simulink model "MRAC_PID_unblance_noposition"  (R2024a)
settings: Solver=FixedStepAuto  StartTime=0.0  StopTime=30  FixedStep=0.001  RelTol=1e-3
values from neighbouring files (symbols this model uses):
  B = [ ... (first row only)    [untitled1.m]
  cM = 2.925e-9    (= 2.925e-09)    [untitled1.m]
  CR = 80.584    [untitled1.m]
  cT = 1.4865e-7    (= 1.4865e-07)    [untitled1.m]
  d_x = 0.08257    [untitled1.m]
  d_y = 0.13505    [untitled1.m]
  g = 9.81    [untitled1.m]
  Ix = 0.0095    [untitled1.m]
  Iy = 0.0095    [untitled1.m]
  Iz = 0.019    [untitled1.m]
  K = cM/cT    (= 0.0196770938446)    [untitled1.m]
  Kposi = 0.1    [untitled1.m]
  Kposp = 1.5    [untitled1.m]
  Kvd = 0    [untitled1.m]
  Kvi = 0    [untitled1.m]
  Kvp = 1    [untitled1.m]
  Kvxd = 10    [untitled1.m]
  Kvxi = 0.001    [untitled1.m]
  Kvxp = 5    [untitled1.m]
  Kvyd = 10    [untitled1.m]
  Kvyi = 0.001    [untitled1.m]
  Kvyp = 5    [untitled1.m]
  Kvzd = 0.1    [untitled1.m]
  Kvzi = 0.01    [untitled1.m]
  Kvzp = 10    [untitled1.m]
  M = inv(B)    [untitled1.m]
  m = 2    [untitled1.m]
  Tm = 0.03    [untitled1.m]
  wb = 976.2    [untitled1.m]
  x1 = d_x    (= 0.08257)    [untitled1.m]
  x2 = d_x    (= 0.08257)    [untitled1.m]
  x3 = -d_x    (= -0.08257)    [untitled1.m]
  x4 = -d_x    (= -0.08257)    [untitled1.m]
  y1 = d_y    (= 0.13505)    [untitled1.m]
  y2 = -d_y    (= -0.13505)    [untitled1.m]
  y3 = -d_y    (= -0.13505)    [untitled1.m]
  y4 = d_y    (= 0.13505)    [untitled1.m]
undefined symbols (not defined in the file or in its folder): magnitude
libraries: slpidlib x5
settings Model: Creator=user  LastModifiedBy=User
settings DataIOCC: ReturnWorkspaceOutputs=off

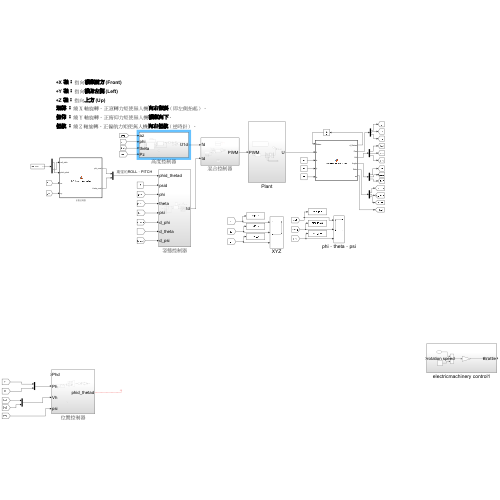
[thumbnail: Simulink's stored preview of the top-level diagram]
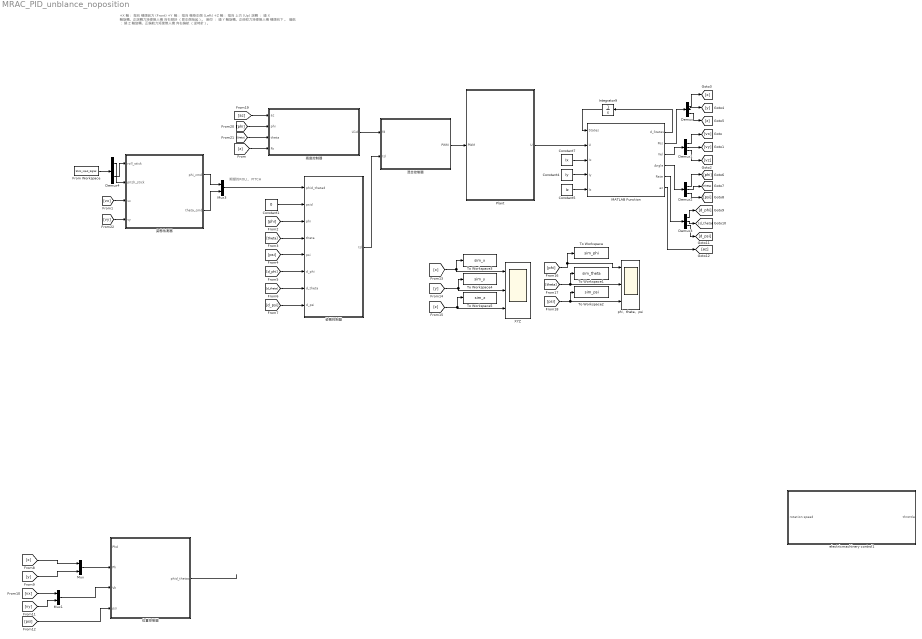
== system MRAC_PID_unblance_noposition ==
  note: +X 軸： 指向 機頭前方 (Front)
      | +Y 軸： 指向 機身左側 (Left)
      | +Z 軸： 指向 上方 (Up)
      | 滾轉 ： 繞 X 軸旋轉。正滾轉力矩使無人機 向右傾斜 （即左側抬起）。
      | 俯仰 ： 繞 Y 軸旋轉。正俯仰力矩使無人機 機頭向下 。
      | 偏航 ： 繞 Z 軸旋轉。正偏航力矩使無人機 向右偏航 （逆時針）。
  note: 期望的ROLL、PITCH
  Constant1 : Constant  Value=0
  Constant4 : Constant  Value=Iy
  Constant5 : Constant  Value=Iz
  Constant7 : Constant  Value=Ix
  Demux{,1..3} (4 alike) : Demux  Outputs=3
  Demux4 : Demux  Outputs=2
  From Workspace : FromWorkspace  VariableName=Stick_Input_Signal
  Integrator9 : Integrator  InitialCondition=zeros(12,1)
  MATLAB Function : MATLAB Function  TreatAsAtomicUnit=on
  Mux : Mux  Inputs=2
  Mux1 : Mux  Inputs=2
  Mux3 : Mux  Inputs=2
  Plant : Subsystem
  To Workspace : ToWorkspace  VariableName=sim_phi  SampleTime=-1
  To Workspace1 : ToWorkspace  VariableName=sim_theta  SampleTime=-1
  To Workspace2 : ToWorkspace  VariableName=sim_psi  SampleTime=-1
  To Workspace3 : ToWorkspace  VariableName=sim_x  SampleTime=-1
  To Workspace4 : ToWorkspace  VariableName=sim_y  SampleTime=-1
  To Workspace5 : ToWorkspace  VariableName=sim_z  SampleTime=-1
  XYZ : Scope  NumInputPorts=3
  electricmachinery control1 : Subsystem
  phi、theta、psi : Scope  NumInputPorts=3
  位置控制器 : Subsystem
  姿態估測器 : MATLAB Function  TreatAsAtomicUnit=on
  姿態控制器 : Subsystem
  混合控制器 : Subsystem
  高度控制器 : Subsystem
  wires:
  高度控制器/1(U1d) -> 混合控制器/1(fd)
  [z] -> 高度控制器/4(Pz)
  位置控制器/1(phid_thetad) -> ?
  Constant1/1 -> 姿態控制器/2(psid)
  [phi] -> 姿態控制器/3(phi)
  [theta] -> 姿態控制器/4(theta)
  [d_psi] -> 姿態控制器/8(d_psi)
  [psi] -> 姿態控制器/5(psi)
  [d_phi] -> 姿態控制器/6(d_phi)
  [d_theta] -> 姿態控制器/7(d_theta)
  姿態控制器/1(td) -> 混合控制器/2(td)
  Mux/1 -> 位置控制器/2(Ph)
  [x] -> Mux/1
  [y] -> Mux/2
  [vx] -> Mux1/1
  [vy] -> Mux1/2
  Mux1/1 -> 位置控制器/3(Vh)
  [psi] -> 位置控制器/4(psi)
  [y] -> To Workspace4/1, XYZ/2
  [x] -> To Workspace3/1, XYZ/1
  [z] -> To Workspace5/1, XYZ/3
  [phi] -> To Workspace/1, phi、theta、psi/1
  [theta] -> To Workspace1/1, phi、theta、psi/2
  [psi] -> To Workspace2/1, phi、theta、psi/3
  混合控制器/1(PWM) -> Plant/1(PWM)
  Constant5/1 -> MATLAB Function/5(Iz)
  Constant7/1 -> MATLAB Function/3(Ix)
  Constant4/1 -> MATLAB Function/4(Iy)
  MATLAB Function/1(d_States) -> Integrator9/1
  Integrator9/1 -> MATLAB Function/1(States)
  MATLAB Function/2(Pos) -> Demux/1
  Demux/1 -> [x]
  Demux/2 -> [y]
  Demux/3 -> [z]
  Demux1/2 -> [vy]
  MATLAB Function/3(Vel) -> Demux1/1
  Demux1/1 -> [vx]
  Demux1/3 -> [vz]
  MATLAB Function/4(Angle) -> Demux2/1
  Demux2/1 -> [phi]
  Demux2/2 -> [theta]
  Demux2/3 -> [psi]
  Demux3/1 -> [d_phi]
  Demux3/2 -> [d_theta]
  Demux3/3 -> [d_psi]
  MATLAB Function/5(Rate) -> Demux3/1
  Plant/1(U) -> MATLAB Function/2(U)
  姿態估測器/1(phi_cmd) -> Mux3/1
  Mux3/1 -> 姿態控制器/1(phid_thetad)
  MATLAB Function/6(az) -> [az]
  [az] -> 高度控制器/1(az)
  [phi] -> 高度控制器/2(phi)
  [theta] -> 高度控制器/3(theta)
  From Workspace/1 -> Demux4/1
  Demux4/1 -> 姿態估測器/2(pitch_stick)
  Demux4/2 -> 姿態估測器/1(roll_stick)
  [vx] -> 姿態估測器/3(vx)
  [vy] -> 姿態估測器/4(vy)
  姿態估測器/2(theta_cmd) -> Mux3/2

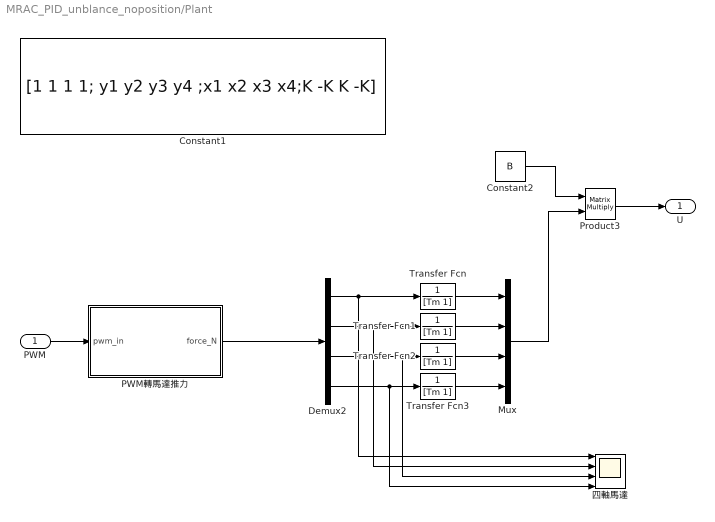
== system MRAC_PID_unblance_noposition/Plant ==
  PWM : Inport
  Constant1 : Constant  Value=[1 1 1 1; y1 y2 y3 y4 ;x1 x2 x3 x4;K -K K -K]
  Constant2 : Constant  Value=B
  Demux2 : Demux
  Mux : Mux
  PWM轉馬達推力 : MATLAB Function  TreatAsAtomicUnit=on
  Product3 : Product  Multiplication=Matrix(*)
  Transfer Fcn{,1..3} (4 alike) : TransferFcn  Denominator=[Tm 1]
  四軸馬達 : Scope  NumInputPorts=4
  U : Outport
  wires:
  Product3/1 -> U/1
  PWM/1 -> PWM轉馬達推力/1(pwm_in)
  Demux2/2 -> Transfer Fcn1/1, 四軸馬達/2
  Demux2/3 -> Transfer Fcn2/1, 四軸馬達/3
  PWM轉馬達推力/1(force_N) -> Demux2/1
  Demux2/4 -> 四軸馬達/4, Transfer Fcn3/1
  Demux2/1 -> Transfer Fcn/1, 四軸馬達/1
  Transfer Fcn1/1 -> Mux/2
  Transfer Fcn/1 -> Mux/1
  Transfer Fcn2/1 -> Mux/3
  Transfer Fcn3/1 -> Mux/4
  Mux/1 -> Product3/2
  Constant2/1 -> Product3/1

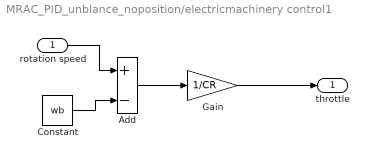
== system MRAC_PID_unblance_noposition/electricmachinery control1 ==
  rotation speed : Inport
  Add : Sum  Inputs=+-
  Constant : Constant  Value=wb
  Gain : Gain  Gain=1/CR
  throttle : Outport
  wires:
  Add/1 -> Gain/1
  rotation speed/1 -> Add/1
  Constant/1 -> Add/2
  Gain/1 -> throttle/1

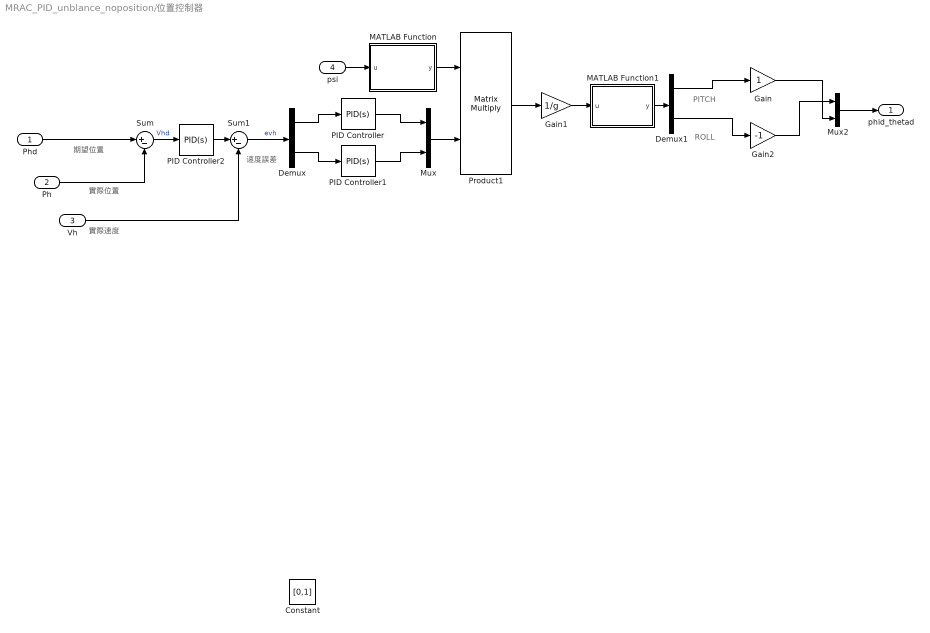
== system MRAC_PID_unblance_noposition/位置控制器 ==
  note: ROLL
  note: 期望位置
  note: 實際位置
  note: 實際速度
  note: 速度誤差
  note: PITCH
  Phd : Inport
  Ph : Inport  Port=2
  Vh : Inport  Port=3
  psi : Inport  Port=4
  Constant : Constant  Value=[0,1]
  Demux : Demux  Outputs=2
  Demux1 : Demux  Outputs=2
  Gain : Gain
  Gain1 : Gain  Gain=1/g
  Gain2 : Gain  Gain=-1
  MATLAB Function : MATLAB Function  TreatAsAtomicUnit=on
  MATLAB Function1 : MATLAB Function  TreatAsAtomicUnit=on
  Mux : Mux  Inputs=2
  Mux2 : Mux  Inputs=2
  PID Controller : slpidlib/PID Controller  Controller=PID  Form=Parallel  TimeDomain=Continuous-time  UseExternalTs=off  SampleTime=-1  IntegratorMethod=Forward Euler  FilterMethod=Forward Euler  ControllerParametersSource=internal  P=Kvxp  I=Kvxi  UseKiTs=off  D=Kvxd  UseExternalDerivativeSource=off  N=100  UseFilter=on  TunerSelectOption=Transfer Function Based (PID Tuner App)  InitialConditionSource=internal  InitialConditionForIntegrator=0  InitialConditionForFilter=0  DifferentiatorICPrevScaledInput=0  ExternalReset=none  TrackingMode=off  Kt=1  LimitOutput=off  SatLimitsSource=internal  UpperSaturationLimit=inf  LowerSaturationLimit=-inf  LinearizeAsGain=on  AntiWindupMode=none  Kb=1  LimitIntegrator=off  UpperIntegratorSaturationLimit=inf  LowerIntegratorSaturationLimit=-inf  POutMin=[]  POutMax=[]  IOutMin=[]  IOutMax=[]  DOutMin=[]  DOutMax=[]  NOutMin=[]  NOutMax=[]  SumOutMin=[]  SumOutMax=[]  SaturationOutMin=[]  SaturationOutMax=[]  PParamMin=[]  PParamMax=[]  IParamMin=[]  IParamMax=[]  DParamMin=[]  DParamMax=[]  NParamMin=[]  NParamMax=[]  KbParamMin=[]  KbParamMax=[]  KtParamMin=[]  KtParamMax=[]  KbOutMin=[]  KbOutMax=[]  KtOutMin=[]  KtOutMax=[]  IntegratorOutMin=[]  IntegratorOutMax=[]  FilterOutMin=[]  FilterOutMax=[]  SumI1OutMin=[]  SumI1OutMax=[]  SumI2OutMin=[]  SumI2OutMax=[]  SumI3OutMin=[]  SumI3OutMax=[]  SumI4OutMin=[]  SumI4OutMax=[]  SumDOutMin=[]  SumDOutMax=[]  DifferentiatorOutMin=[]  DifferentiatorOutMax=[]  FilterDiffOutCoefMin=[]  FilterDiffOutCoefMax=[]  ReciprocalOutMin=[]  ReciprocalOutMax=[]  SumDenOutMin=[]  SumDenOutMax=[]  SumNumOutMin=[]  SumNumOutMax=[]  DivideOutMin=[]  DivideOutMax=[]  UdiffTsProdOutMin=[]  UdiffTsProdOutMax=[]  NTsProdOutMin=[]  NTsProdOutMax=[]  UintegralTsProdOutMin=[]  UintegralTsProdOutMax=[]  UngainTsProdOutMin=[]  UngainTsProdOutMax=[]  ClampingZeroOutDataTypeStr=Inherit: Inherit via back propagation  ClampingZeroOutMin=[]  ClampingZeroOutMax=[]  FilterDenConstantOutDataTypeStr=Inherit: Inherit via back propagation  FilterDenConstantOutMin=[]  FilterDenConstantOutMax=[]  PCopyOutDataTypeStr=Inherit: Inherit via back propagation  PCopyOutMin=[]  PCopyOutMax=[]  NCopyOutDataTypeStr=Inherit: Inherit via back propagation  NCopyOutMin=[]  NCopyOutMax=[]  IntegratorContinuousStateAttributes=''  IntegratorStateMustResolveToSignalObject=off  IntegratorRTWStateStorageClass=Auto  FilterContinuousStateAttributes=''  FilterStateMustResolveToSignalObject=off  FilterRTWStateStorageClass=Auto  ParallelPVariant=InternalParameters  IdealPVariant=Disabled  IVariant=InternalParameters  DVariant=InternalParameters  IntegratorVariant=Continuous  SatVariant=Disabled  AWVariant=Passthrough  PCopyVariant=Disabled  TRVariant=Disabled  FdbkBlocksVariant=Forward  IdealPFdbkVariant=Disabled  SatFdbkVariant=Disabled  DerivativeFilterVariant=ContFilter  NVariant=InternalParameters  NCopyVariant=Disabled  FilterICVariant=InternalICsFilter  IntegratorICVariant=InternalICs  ExternalResetVariant=Disabled  TRSumVariant=Passthrough  SumFdbkVariant=Disabled  SumVariant=Sum_PID  TsampFilterVariant=InternalTs  TsampNgainVariant=Passthrough  TsampIntegralVariant=Disabled_SignalSpec  ExternalSaturationOutDataTypeStr=Inherit: Same as second input  DerivativeSourceVariant=ErrorSignal
  PID Controller1 : slpidlib/PID Controller  Controller=PID  Form=Parallel  TimeDomain=Continuous-time  UseExternalTs=off  SampleTime=-1  IntegratorMethod=Forward Euler  FilterMethod=Forward Euler  ControllerParametersSource=internal  P=Kvyp  I=Kvyi  UseKiTs=off  D=Kvyd  UseExternalDerivativeSource=off  N=100  UseFilter=on  TunerSelectOption=Transfer Function Based (PID Tuner App)  InitialConditionSource=internal  InitialConditionForIntegrator=0  InitialConditionForFilter=0  DifferentiatorICPrevScaledInput=0  ExternalReset=none  TrackingMode=off  Kt=1  LimitOutput=off  SatLimitsSource=internal  UpperSaturationLimit=inf  LowerSaturationLimit=-inf  LinearizeAsGain=on  AntiWindupMode=none  Kb=1  LimitIntegrator=off  UpperIntegratorSaturationLimit=inf  LowerIntegratorSaturationLimit=-inf  POutMin=[]  POutMax=[]  IOutMin=[]  IOutMax=[]  DOutMin=[]  DOutMax=[]  NOutMin=[]  NOutMax=[]  SumOutMin=[]  SumOutMax=[]  SaturationOutMin=[]  SaturationOutMax=[]  PParamMin=[]  PParamMax=[]  IParamMin=[]  IParamMax=[]  DParamMin=[]  DParamMax=[]  NParamMin=[]  NParamMax=[]  KbParamMin=[]  KbParamMax=[]  KtParamMin=[]  KtParamMax=[]  KbOutMin=[]  KbOutMax=[]  KtOutMin=[]  KtOutMax=[]  IntegratorOutMin=[]  IntegratorOutMax=[]  FilterOutMin=[]  FilterOutMax=[]  SumI1OutMin=[]  SumI1OutMax=[]  SumI2OutMin=[]  SumI2OutMax=[]  SumI3OutMin=[]  SumI3OutMax=[]  SumI4OutMin=[]  SumI4OutMax=[]  SumDOutMin=[]  SumDOutMax=[]  DifferentiatorOutMin=[]  DifferentiatorOutMax=[]  FilterDiffOutCoefMin=[]  FilterDiffOutCoefMax=[]  ReciprocalOutMin=[]  ReciprocalOutMax=[]  SumDenOutMin=[]  SumDenOutMax=[]  SumNumOutMin=[]  SumNumOutMax=[]  DivideOutMin=[]  DivideOutMax=[]  UdiffTsProdOutMin=[]  UdiffTsProdOutMax=[]  NTsProdOutMin=[]  NTsProdOutMax=[]  UintegralTsProdOutMin=[]  UintegralTsProdOutMax=[]  UngainTsProdOutMin=[]  UngainTsProdOutMax=[]  ClampingZeroOutDataTypeStr=Inherit: Inherit via back propagation  ClampingZeroOutMin=[]  ClampingZeroOutMax=[]  FilterDenConstantOutDataTypeStr=Inherit: Inherit via back propagation  FilterDenConstantOutMin=[]  FilterDenConstantOutMax=[]  PCopyOutDataTypeStr=Inherit: Inherit via back propagation  PCopyOutMin=[]  PCopyOutMax=[]  NCopyOutDataTypeStr=Inherit: Inherit via back propagation  NCopyOutMin=[]  NCopyOutMax=[]  IntegratorContinuousStateAttributes=''  IntegratorStateMustResolveToSignalObject=off  IntegratorRTWStateStorageClass=Auto  FilterContinuousStateAttributes=''  FilterStateMustResolveToSignalObject=off  FilterRTWStateStorageClass=Auto  ParallelPVariant=InternalParameters  IdealPVariant=Disabled  IVariant=InternalParameters  DVariant=InternalParameters  IntegratorVariant=Continuous  SatVariant=Disabled  AWVariant=Passthrough  PCopyVariant=Disabled  TRVariant=Disabled  FdbkBlocksVariant=Forward  IdealPFdbkVariant=Disabled  SatFdbkVariant=Disabled  DerivativeFilterVariant=ContFilter  NVariant=InternalParameters  NCopyVariant=Disabled  FilterICVariant=InternalICsFilter  IntegratorICVariant=InternalICs  ExternalResetVariant=Disabled  TRSumVariant=Passthrough  SumFdbkVariant=Disabled  SumVariant=Sum_PID  TsampFilterVariant=InternalTs  TsampNgainVariant=Passthrough  TsampIntegralVariant=Disabled_SignalSpec  ExternalSaturationOutDataTypeStr=Inherit: Same as second input  DerivativeSourceVariant=ErrorSignal
  PID Controller2 : slpidlib/PID Controller  Controller=PID  Form=Parallel  TimeDomain=Continuous-time  UseExternalTs=off  SampleTime=-1  IntegratorMethod=Forward Euler  FilterMethod=Forward Euler  ControllerParametersSource=internal  P=Kposp  I=Kposi  UseKiTs=off  D=0  UseExternalDerivativeSource=off  N=100  UseFilter=on  TunerSelectOption=Transfer Function Based (PID Tuner App)  InitialConditionSource=internal  InitialConditionForIntegrator=0  InitialConditionForFilter=0  DifferentiatorICPrevScaledInput=0  ExternalReset=none  TrackingMode=off  Kt=1  LimitOutput=off  SatLimitsSource=internal  UpperSaturationLimit=inf  LowerSaturationLimit=-inf  LinearizeAsGain=on  AntiWindupMode=none  Kb=1  LimitIntegrator=off  UpperIntegratorSaturationLimit=inf  LowerIntegratorSaturationLimit=-inf  POutMin=[]  POutMax=[]  IOutMin=[]  IOutMax=[]  DOutMin=[]  DOutMax=[]  NOutMin=[]  NOutMax=[]  SumOutMin=[]  SumOutMax=[]  SaturationOutMin=[]  SaturationOutMax=[]  PParamMin=[]  PParamMax=[]  IParamMin=[]  IParamMax=[]  DParamMin=[]  DParamMax=[]  NParamMin=[]  NParamMax=[]  KbParamMin=[]  KbParamMax=[]  KtParamMin=[]  KtParamMax=[]  KbOutMin=[]  KbOutMax=[]  KtOutMin=[]  KtOutMax=[]  IntegratorOutMin=[]  IntegratorOutMax=[]  FilterOutMin=[]  FilterOutMax=[]  SumI1OutMin=[]  SumI1OutMax=[]  SumI2OutMin=[]  SumI2OutMax=[]  SumI3OutMin=[]  SumI3OutMax=[]  SumI4OutMin=[]  SumI4OutMax=[]  SumDOutMin=[]  SumDOutMax=[]  DifferentiatorOutMin=[]  DifferentiatorOutMax=[]  FilterDiffOutCoefMin=[]  FilterDiffOutCoefMax=[]  ReciprocalOutMin=[]  ReciprocalOutMax=[]  SumDenOutMin=[]  SumDenOutMax=[]  SumNumOutMin=[]  SumNumOutMax=[]  DivideOutMin=[]  DivideOutMax=[]  UdiffTsProdOutMin=[]  UdiffTsProdOutMax=[]  NTsProdOutMin=[]  NTsProdOutMax=[]  UintegralTsProdOutMin=[]  UintegralTsProdOutMax=[]  UngainTsProdOutMin=[]  UngainTsProdOutMax=[]  ClampingZeroOutDataTypeStr=Inherit: Inherit via back propagation  ClampingZeroOutMin=[]  ClampingZeroOutMax=[]  FilterDenConstantOutDataTypeStr=Inherit: Inherit via back propagation  FilterDenConstantOutMin=[]  FilterDenConstantOutMax=[]  PCopyOutDataTypeStr=Inherit: Inherit via back propagation  PCopyOutMin=[]  PCopyOutMax=[]  NCopyOutDataTypeStr=Inherit: Inherit via back propagation  NCopyOutMin=[]  NCopyOutMax=[]  IntegratorContinuousStateAttributes=''  IntegratorStateMustResolveToSignalObject=off  IntegratorRTWStateStorageClass=Auto  FilterContinuousStateAttributes=''  FilterStateMustResolveToSignalObject=off  FilterRTWStateStorageClass=Auto  ParallelPVariant=InternalParameters  IdealPVariant=Disabled  IVariant=InternalParameters  DVariant=InternalParameters  IntegratorVariant=Continuous  SatVariant=Disabled  AWVariant=Passthrough  PCopyVariant=Disabled  TRVariant=Disabled  FdbkBlocksVariant=Forward  IdealPFdbkVariant=Disabled  SatFdbkVariant=Disabled  DerivativeFilterVariant=ContFilter  NVariant=InternalParameters  NCopyVariant=Disabled  FilterICVariant=InternalICsFilter  IntegratorICVariant=InternalICs  ExternalResetVariant=Disabled  TRSumVariant=Passthrough  SumFdbkVariant=Disabled  SumVariant=Sum_PID  TsampFilterVariant=InternalTs  TsampNgainVariant=Passthrough  TsampIntegralVariant=Disabled_SignalSpec  ExternalSaturationOutDataTypeStr=Inherit: Same as second input  DerivativeSourceVariant=ErrorSignal
  Product1 : Product  Multiplication=Matrix(*)
  Sum : Sum  Inputs=|+-
  Sum1 : Sum  Inputs=|+-
  phid_thetad : Outport
  wires:
  Gain1/1 -> MATLAB Function1/1(u)
  Demux/1 -> PID Controller/1
  Product1/1 -> Gain1/1
  PID Controller/1 -> Mux/1
  Demux/2 -> PID Controller1/1
  Sum1/1 -> Demux/1  "evh"
  Mux/1 -> Product1/2
  Sum/1 -> PID Controller2/1  "Vhd"
  MATLAB Function1/1(y) -> Demux1/1
  MATLAB Function/1(y) -> Product1/1
  PID Controller1/1 -> Mux/2
  Demux1/1 -> Gain/1
  Gain/1 -> Mux2/2
  Mux2/1 -> phid_thetad/1
  Ph/1 -> Sum/2
  Phd/1 -> Sum/1
  PID Controller2/1 -> Sum1/1
  Vh/1 -> Sum1/2
  Demux1/2 -> Gain2/1
  psi/1 -> MATLAB Function/1(u)
  Gain2/1 -> Mux2/1

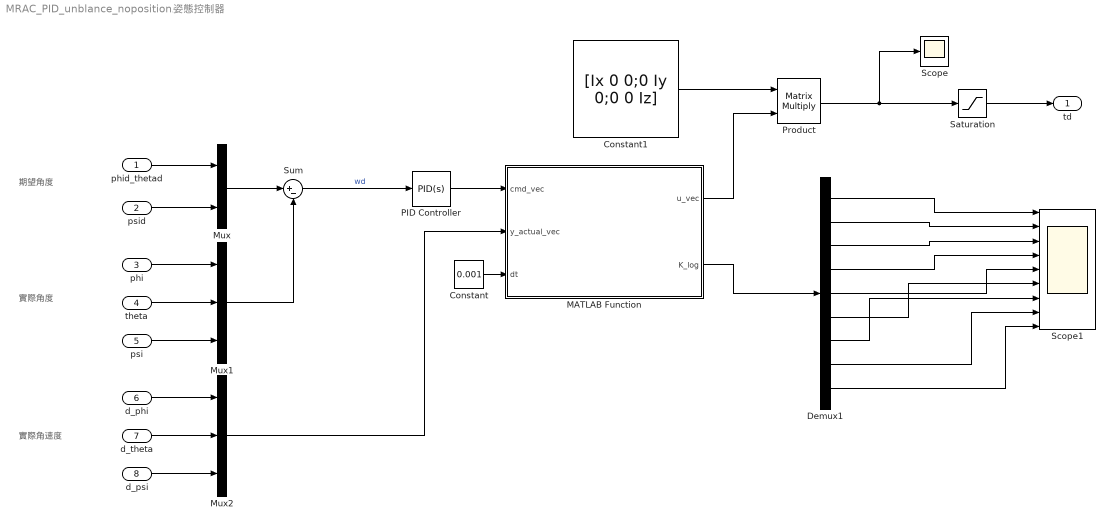
== system MRAC_PID_unblance_noposition/姿態控制器 ==
  note: 實際角速度
  note: 實際角度
  note: 期望角度
  phid_thetad : Inport
  psid : Inport  Port=2
  phi : Inport  Port=3
  theta : Inport  Port=4
  psi : Inport  Port=5
  d_phi : Inport  Port=6
  d_theta : Inport  Port=7
  d_psi : Inport  Port=8
  Constant : Constant  Value=0.001
  Constant1 : Constant  Value=[Ix 0 0;0 Iy 0;0 0 Iz]
  Demux1 : Demux  Outputs=9
  MATLAB Function : MATLAB Function  TreatAsAtomicUnit=on
  Mux : Mux  Inputs=2
  Mux1 : Mux  Inputs=3
  Mux2 : Mux  Inputs=3
  PID Controller : slpidlib/PID Controller  Controller=PID  Form=Parallel  TimeDomain=Continuous-time  UseExternalTs=off  SampleTime=-1  IntegratorMethod=Forward Euler  FilterMethod=Forward Euler  ControllerParametersSource=internal  P=Kvp  I=Kvi  UseKiTs=off  D=Kvd  UseExternalDerivativeSource=off  N=100  UseFilter=on  TunerSelectOption=Transfer Function Based (PID Tuner App)  InitialConditionSource=internal  InitialConditionForIntegrator=0  InitialConditionForFilter=0  DifferentiatorICPrevScaledInput=0  ExternalReset=none  TrackingMode=off  Kt=1  LimitOutput=off  SatLimitsSource=internal  UpperSaturationLimit=inf  LowerSaturationLimit=-inf  LinearizeAsGain=on  AntiWindupMode=none  Kb=1  LimitIntegrator=off  UpperIntegratorSaturationLimit=inf  LowerIntegratorSaturationLimit=-inf  POutMin=[]  POutMax=[]  IOutMin=[]  IOutMax=[]  DOutMin=[]  DOutMax=[]  NOutMin=[]  NOutMax=[]  SumOutMin=[]  SumOutMax=[]  SaturationOutMin=[]  SaturationOutMax=[]  PParamMin=[]  PParamMax=[]  IParamMin=[]  IParamMax=[]  DParamMin=[]  DParamMax=[]  NParamMin=[]  NParamMax=[]  KbParamMin=[]  KbParamMax=[]  KtParamMin=[]  KtParamMax=[]  KbOutMin=[]  KbOutMax=[]  KtOutMin=[]  KtOutMax=[]  IntegratorOutMin=[]  IntegratorOutMax=[]  FilterOutMin=[]  FilterOutMax=[]  SumI1OutMin=[]  SumI1OutMax=[]  SumI2OutMin=[]  SumI2OutMax=[]  SumI3OutMin=[]  SumI3OutMax=[]  SumI4OutMin=[]  SumI4OutMax=[]  SumDOutMin=[]  SumDOutMax=[]  DifferentiatorOutMin=[]  DifferentiatorOutMax=[]  FilterDiffOutCoefMin=[]  FilterDiffOutCoefMax=[]  ReciprocalOutMin=[]  ReciprocalOutMax=[]  SumDenOutMin=[]  SumDenOutMax=[]  SumNumOutMin=[]  SumNumOutMax=[]  DivideOutMin=[]  DivideOutMax=[]  UdiffTsProdOutMin=[]  UdiffTsProdOutMax=[]  NTsProdOutMin=[]  NTsProdOutMax=[]  UintegralTsProdOutMin=[]  UintegralTsProdOutMax=[]  UngainTsProdOutMin=[]  UngainTsProdOutMax=[]  ClampingZeroOutDataTypeStr=Inherit: Inherit via back propagation  ClampingZeroOutMin=[]  ClampingZeroOutMax=[]  FilterDenConstantOutDataTypeStr=Inherit: Inherit via back propagation  FilterDenConstantOutMin=[]  FilterDenConstantOutMax=[]  PCopyOutDataTypeStr=Inherit: Inherit via back propagation  PCopyOutMin=[]  PCopyOutMax=[]  NCopyOutDataTypeStr=Inherit: Inherit via back propagation  NCopyOutMin=[]  NCopyOutMax=[]  IntegratorContinuousStateAttributes=''  IntegratorStateMustResolveToSignalObject=off  IntegratorRTWStateStorageClass=Auto  FilterContinuousStateAttributes=''  FilterStateMustResolveToSignalObject=off  FilterRTWStateStorageClass=Auto  ParallelPVariant=InternalParameters  IdealPVariant=Disabled  IVariant=InternalParameters  DVariant=InternalParameters  IntegratorVariant=Continuous  SatVariant=Disabled  AWVariant=Passthrough  PCopyVariant=Disabled  TRVariant=Disabled  FdbkBlocksVariant=Forward  IdealPFdbkVariant=Disabled  SatFdbkVariant=Disabled  DerivativeFilterVariant=ContFilter  NVariant=InternalParameters  NCopyVariant=Disabled  FilterICVariant=InternalICsFilter  IntegratorICVariant=InternalICs  ExternalResetVariant=Disabled  TRSumVariant=Passthrough  SumFdbkVariant=Disabled  SumVariant=Sum_PID  TsampFilterVariant=InternalTs  TsampNgainVariant=Passthrough  TsampIntegralVariant=Disabled_SignalSpec  ExternalSaturationOutDataTypeStr=Inherit: Same as second input  DerivativeSourceVariant=ErrorSignal
  Product : Product  Multiplication=Matrix(*)
  Saturation : Saturate  UpperLimit=0.7  LowerLimit=-0.7
  Scope : Scope
  Scope1 : Scope  NumInputPorts=9
  Sum : Sum  Inputs=|+-
  td : Outport
  wires:
  phid_thetad/1 -> Mux/1
  phi/1 -> Mux1/1
  psid/1 -> Mux/2
  theta/1 -> Mux1/2
  Mux1/1 -> Sum/2
  d_psi/1 -> Mux2/3
  Constant1/1 -> Product/1
  d_theta/1 -> Mux2/2
  Sum/1 -> PID Controller/1  "wd"
  Constant/1 -> MATLAB Function/3(dt)
  d_phi/1 -> Mux2/1
  MATLAB Function/1(u_vec) -> Product/2
  MATLAB Function/2(K_log) -> Demux1/1
  psi/1 -> Mux1/3
  Mux/1 -> Sum/1
  Mux2/1 -> MATLAB Function/2(y_actual_vec)
  Product/1 -> Scope/1, Saturation/1
  Saturation/1 -> td/1
  PID Controller/1 -> MATLAB Function/1(cmd_vec)
  Demux1/1 -> Scope1/1
  Demux1/2 -> Scope1/2
  Demux1/3 -> Scope1/3
  Demux1/4 -> Scope1/4
  Demux1/5 -> Scope1/5
  Demux1/6 -> Scope1/6
  Demux1/7 -> Scope1/7
  Demux1/8 -> Scope1/8
  Demux1/9 -> Scope1/9

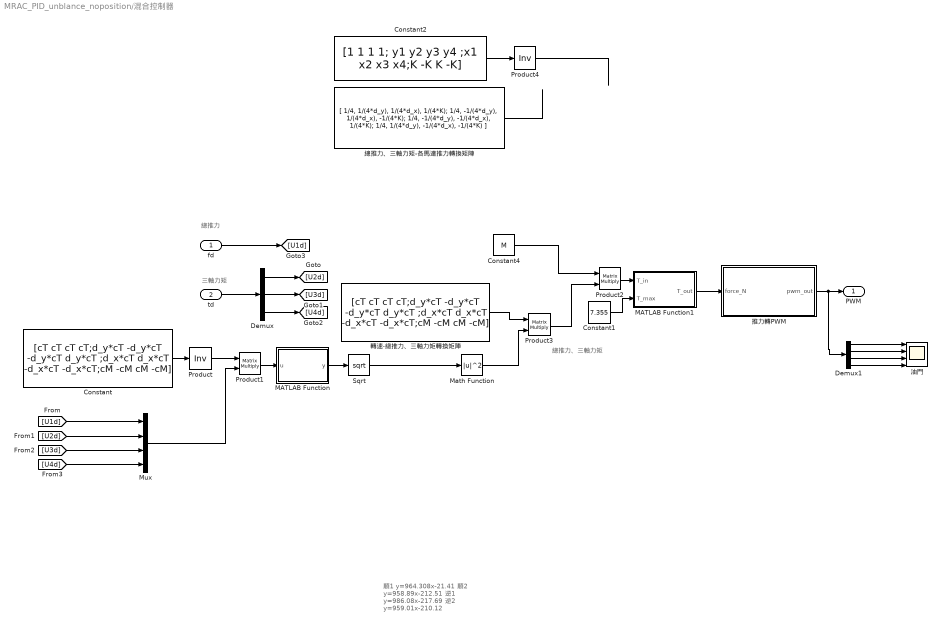
== system MRAC_PID_unblance_noposition/混合控制器 ==
  note: 三軸力矩
  note: 總推力
  note: 總推力、三軸力矩
  note: 順1 y=964.308x-21.41
      | 順2 y=958.89x-212.51
      | 逆1 y=986.08x-217.69
      | 逆2 y=959.01x-210.12
  fd : Inport
  td : Inport  Port=2
  Constant : Constant  Value=[cT cT cT cT;d_y*cT -d_y*cT -d_y*cT d_y*cT ;d_x*cT d_x*cT -d_x*cT -d_x*cT;cM -cM cM -cM]
  Constant1 : Constant  Value=7.355
  Constant2 : Constant  Value=[1 1 1 1; y1 y2 y3 y4 ;x1 x2 x3 x4;K -K K -K]
  Constant4 : Constant  Value=M
  Demux : Demux  Outputs=3
  Demux1 : Demux
  MATLAB Function : MATLAB Function  TreatAsAtomicUnit=on
  MATLAB Function1 : MATLAB Function  TreatAsAtomicUnit=on
  Math Function : Math  Operator=magnitude^2
  Mux : Mux
  Product : Product  Inputs=/  Multiplication=Matrix(*)
  Product1 : Product  Multiplication=Matrix(*)
  Product2 : Product  Multiplication=Matrix(*)
  Product3 : Product  Multiplication=Matrix(*)
  Product4 : Product  Inputs=/  Multiplication=Matrix(*)
  Sqrt : Sqrt
  推力轉PWM : MATLAB Function  TreatAsAtomicUnit=on
  油門 : Scope  NumInputPorts=4
  總推力、三軸力矩-各馬達推力轉換矩陣 : Constant  Value=|
      | [ 1/4,    1/(4*d_y),    1/(4*d_x),    1/(4*K);
      |   1/4,   -1/(4*d_y),    1/(4*d_x),   -1/(4*K);
      |   1/4,   -1/(4*d_y),   -1/(4*d_x),    1/(4*K);
      |   1/4,    1/(4*d_y),   -1/(4*d_x),   -1/(4*K) ]
  轉速-總推力、三軸力矩轉換矩陣 : Constant  Value=[cT cT cT cT;d_y*cT -d_y*cT -d_y*cT d_y*cT ;d_x*cT d_x*cT -d_x*cT -d_x*cT;cM -cM cM -cM]
  PWM : Outport
  wires:
  [U4d] -> Mux/4
  td/1 -> Demux/1
  Constant/1 -> Product/1
  Mux/1 -> Product1/2
  Demux/1 -> [U2d]
  [U3d] -> Mux/3
  [U2d] -> Mux/2
  Product/1 -> Product1/1
  fd/1 -> [U1d]
  Demux/3 -> [U4d]
  Demux/2 -> [U3d]
  [U1d] -> Mux/1
  Product1/1 -> MATLAB Function/1(u)
  MATLAB Function/1(y) -> Sqrt/1
  Product3/1 -> Product2/2
  轉速-總推力、三軸力矩轉換矩陣/1 -> Product3/1
  Sqrt/1 -> Math Function/1
  Product2/1 -> MATLAB Function1/1(T_in)
  MATLAB Function1/1(T_out) -> 推力轉PWM/1(force_N)
  Constant1/1 -> MATLAB Function1/2(T_max)
  Math Function/1 -> Product3/2
  總推力、三軸力矩-各馬達推力轉換矩陣/1 -> ?
  推力轉PWM/1(pwm_out) -> Demux1/1, PWM/1
  Demux1/1 -> 油門/1
  Demux1/2 -> 油門/2
  Demux1/3 -> 油門/3
  Demux1/4 -> 油門/4
  Constant2/1 -> Product4/1
  Product4/1 -> ?
  Constant4/1 -> Product2/1

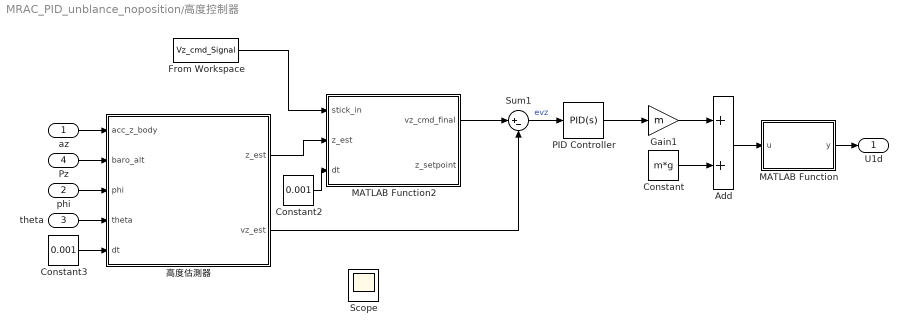
== system MRAC_PID_unblance_noposition/高度控制器 ==
  az : Inport
  phi : Inport  Port=2
  theta : Inport  Port=3
  Pz : Inport  Port=4
  Add : Sum
  Constant : Constant  Value=m*g
  Constant2 : Constant  Value=0.001
  Constant3 : Constant  Value=0.001
  From Workspace : FromWorkspace  VariableName=Vz_cmd_Signal
  Gain1 : Gain  Gain=m
  MATLAB Function : MATLAB Function  TreatAsAtomicUnit=on
  MATLAB Function2 : MATLAB Function  TreatAsAtomicUnit=on
  PID Controller : slpidlib/PID Controller  Controller=PID  Form=Parallel  TimeDomain=Continuous-time  UseExternalTs=off  SampleTime=-1  IntegratorMethod=Forward Euler  FilterMethod=Forward Euler  ControllerParametersSource=internal  P=Kvzp  I=Kvzi  UseKiTs=off  D=Kvzd  UseExternalDerivativeSource=off  N=100  UseFilter=on  TunerSelectOption=Transfer Function Based (PID Tuner App)  InitialConditionSource=internal  InitialConditionForIntegrator=0  InitialConditionForFilter=0  DifferentiatorICPrevScaledInput=0  ExternalReset=none  TrackingMode=off  Kt=1  LimitOutput=on  SatLimitsSource=internal  UpperSaturationLimit=29.42  LowerSaturationLimit=-29.42  LinearizeAsGain=on  AntiWindupMode=none  Kb=1  LimitIntegrator=off  UpperIntegratorSaturationLimit=inf  LowerIntegratorSaturationLimit=-inf  POutMin=[]  POutMax=[]  IOutMin=[]  IOutMax=[]  DOutMin=[]  DOutMax=[]  NOutMin=[]  NOutMax=[]  SumOutMin=[]  SumOutMax=[]  SaturationOutMin=[]  SaturationOutMax=[]  PParamMin=[]  PParamMax=[]  IParamMin=[]  IParamMax=[]  DParamMin=[]  DParamMax=[]  NParamMin=[]  NParamMax=[]  KbParamMin=[]  KbParamMax=[]  KtParamMin=[]  KtParamMax=[]  KbOutMin=[]  KbOutMax=[]  KtOutMin=[]  KtOutMax=[]  IntegratorOutMin=[]  IntegratorOutMax=[]  FilterOutMin=[]  FilterOutMax=[]  SumI1OutMin=[]  SumI1OutMax=[]  SumI2OutMin=[]  SumI2OutMax=[]  SumI3OutMin=[]  SumI3OutMax=[]  SumI4OutMin=[]  SumI4OutMax=[]  SumDOutMin=[]  SumDOutMax=[]  DifferentiatorOutMin=[]  DifferentiatorOutMax=[]  FilterDiffOutCoefMin=[]  FilterDiffOutCoefMax=[]  ReciprocalOutMin=[]  ReciprocalOutMax=[]  SumDenOutMin=[]  SumDenOutMax=[]  SumNumOutMin=[]  SumNumOutMax=[]  DivideOutMin=[]  DivideOutMax=[]  UdiffTsProdOutMin=[]  UdiffTsProdOutMax=[]  NTsProdOutMin=[]  NTsProdOutMax=[]  UintegralTsProdOutMin=[]  UintegralTsProdOutMax=[]  UngainTsProdOutMin=[]  UngainTsProdOutMax=[]  ClampingZeroOutDataTypeStr=Inherit: Inherit via back propagation  ClampingZeroOutMin=[]  ClampingZeroOutMax=[]  FilterDenConstantOutDataTypeStr=Inherit: Inherit via back propagation  FilterDenConstantOutMin=[]  FilterDenConstantOutMax=[]  PCopyOutDataTypeStr=Inherit: Inherit via back propagation  PCopyOutMin=[]  PCopyOutMax=[]  NCopyOutDataTypeStr=Inherit: Inherit via back propagation  NCopyOutMin=[]  NCopyOutMax=[]  IntegratorContinuousStateAttributes=''  IntegratorStateMustResolveToSignalObject=off  IntegratorRTWStateStorageClass=Auto  FilterContinuousStateAttributes=''  FilterStateMustResolveToSignalObject=off  FilterRTWStateStorageClass=Auto  ParallelPVariant=InternalParameters  IdealPVariant=Disabled  IVariant=InternalParameters  DVariant=InternalParameters  IntegratorVariant=Continuous  SatVariant=Enabled  AWVariant=Passthrough  PCopyVariant=Disabled  TRVariant=Disabled  FdbkBlocksVariant=Forward  IdealPFdbkVariant=Disabled  SatFdbkVariant=Disabled  DerivativeFilterVariant=ContFilter  NVariant=InternalParameters  NCopyVariant=Disabled  FilterICVariant=InternalICsFilter  IntegratorICVariant=InternalICs  ExternalResetVariant=Disabled  TRSumVariant=Passthrough  SumFdbkVariant=Disabled  SumVariant=Sum_PID  TsampFilterVariant=InternalTs  TsampNgainVariant=Passthrough  TsampIntegralVariant=Disabled_SignalSpec  ExternalSaturationOutDataTypeStr=Inherit: Same as second input  DerivativeSourceVariant=ErrorSignal
  Scope : Scope
  Sum1 : Sum  Inputs=|+-
  高度估測器 : MATLAB Function  TreatAsAtomicUnit=on
  U1d : Outport
  wires:
  PID Controller/1 -> Gain1/1
  Sum1/1 -> PID Controller/1  "evz"
  Pz/1 -> 高度估測器/2(baro_alt)
  Gain1/1 -> Add/1
  Constant/1 -> Add/2
  MATLAB Function/1(y) -> U1d/1
  Add/1 -> MATLAB Function/1(u)
  From Workspace/1 -> MATLAB Function2/1(stick_in)
  MATLAB Function2/1(vz_cmd_final) -> Sum1/1
  高度估測器/1(z_est) -> MATLAB Function2/2(z_est)
  Constant2/1 -> MATLAB Function2/3(dt)
  az/1 -> 高度估測器/1(acc_z_body)
  Constant3/1 -> 高度估測器/5(dt)
  phi/1 -> 高度估測器/3(phi)
  theta/1 -> 高度估測器/4(theta)
  高度估測器/2(vz_est) -> Sum1/2

== matlab function MRAC_PID_unblance_noposition/高度控制器/高度估測器 ==
  settings: updateMethod=DISCRETE
  data: acc_z_body input; z_est output; baro_alt input; phi input; theta input; dt input; vz_est output
function [z_est, vz_est] = fcn(acc_z_body, baro_alt, phi, theta, dt)


    persistent z_hat vz_hat
    if isempty(z_hat)
        z_hat = baro_alt;   % 初始高度
        vz_hat = 0;
    end
    
    % 1. 座標轉換
    g = 9.81;
    acc_z_earth = acc_z_body * cos(phi) * cos(theta) ;
    
    % 2. 互補濾波
    K_z_obs = 2.0;   
    K_vz_obs = 0.2;

    % 預測
    z_predict = z_hat + vz_hat * dt;
    vz_predict = vz_hat + acc_z_earth * dt;
    
    % 誤差
    z_err = baro_alt - z_predict;
    
    % 校正
    z_est = z_predict + K_z_obs * z_err * dt;
    vz_est = vz_predict + K_vz_obs * z_err * dt;
    
    % 更新狀態
    z_hat = z_est;
    vz_hat = vz_est;
end

== matlab function MRAC_PID_unblance_noposition/高度控制器/MATLAB Function2 ==
  settings: updateMethod=DISCRETE
  data: stick_in input; vz_cmd_final output; z_est input; dt input; z_setpoint output
function [vz_cmd_final, z_setpoint] = Alt_Logic_Controller(stick_in, z_est, dt)


    % 參數
    deadzone = 0.1;      % 搖桿死區
    max_climb_rate = 2.0; % 最大速度
    Kp_z_outer = 1.0;    % 外層位置控制器的 P 增益
    
    % 狀態記憶
    persistent z_lock_target 
    
    if isempty(z_lock_target)
        z_lock_target = 0;
    end
    
   
    if abs(stick_in) > deadzone
        vz_cmd_final = stick_in * max_climb_rate;
        z_lock_target = z_est;
    else
        pos_error = z_lock_target - z_est;
        vz_correction = pos_error * Kp_z_outer;

        if vz_correction > max_climb_rate
            vz_correction = max_climb_rate;
        elseif vz_correction < -max_climb_rate
            vz_correction = -max_climb_rate;
        end
        
        vz_cmd_final = vz_correction;
    end
    z_setpoint = z_lock_target;
    
end

== matlab function MRAC_PID_unblance_noposition/高度控制器/MATLAB Function ==
  data: u input; y output
function y = fcn(u)
u(u>29.42) = 29.42;
y = u;

== matlab function MRAC_PID_unblance_noposition/混合控制器/MATLAB Function ==
  data: u input; y output
function y = fcn(u)
u(u<0) = 0;
y = u;

== matlab function MRAC_PID_unblance_noposition/位置控制器/MATLAB Function ==
  data: u input; y output
function y = fcn(u)
 
y = [cos(u) sin(u);
     -sin(u) cos(u)];

% y = [sin(u) cos(u);
%      -cos(u) sin(u)];

== matlab function MRAC_PID_unblance_noposition/位置控制器/MATLAB Function1 ==
  data: u input; y output
function y = fcn(u)
u(u>0.5) = 0.5;
u(u<-0.5) = -0.5;
y = u;

== matlab function MRAC_PID_unblance_noposition/混合控制器/MATLAB Function1 ==
  data: T_in input; T_out output; T_max input
function T_out = fcn(T_in, T_max)

% 1. 找出四個馬達中，需求最大的那個值
max_thrust_req = max(T_in);

% 2. 計算超出的量
excess = max_thrust_req - T_max;

% 3. 動態飽和邏輯
if excess > 0
    T_out = T_in - excess;
else

    T_out = T_in;
end

% 4. 下限保護
for i = 1:4
    if T_out(i) < 0
        T_out(i) = 0;
    end
end

% 5. 再次上限保護
for i = 1:4
    if T_out(i) > T_max
        T_out(i) = T_max;
    end
end

== matlab function MRAC_PID_unblance_noposition/姿態控制器/MATLAB Function ==
  settings: updateMethod=DISCRETE
  data: cmd_vec input; u_vec output; y_actual_vec input; dt input; K_log output
function [u_vec, K_log] = fcn_MRAC_3Axis(cmd_vec, y_actual_vec, dt)
    % A. 參考模型
    wn_vec   = [10;  5;   5];    
    zeta_vec = [0.707; 0.707; 0.707];
    
    % B. 自適應增益
    % gam_p_vec = [0.01; 0.01; 0.01]; 
    % gam_i_vec = [0.01; 0.01; 0.01];
    % gam_d_vec = [0.001; 0.001; 0.001];

    gam_p_vec = [1;1; 1]; 
    gam_i_vec = [1;1; 1];
    gam_d_vec = [0.01;0.01; 0.01];
    
    % C. PID 初始值
    Kp_init = [1000; 1000;  20];
    Ki_init = [50;  50;  0.1];
    Kd_init = [10;  10;  5];
    
    % D. 參數限制
    Kp_max = [10000; 10000; 10000]; Kp_min = [0.01; 0.01; 0.01];
    Ki_max = [10000; 10000; 10000]; Ki_min = [0; 0; 0];
    Kd_max = [1000;  1000;  500];  Kd_min = [0; 0; 0];

 
    persistent xm_1 xm_2        % 參考模型狀態
    persistent e_integral       % 積分誤差
    persistent prev_error       % 上一次誤差
    persistent Kp Ki Kd         % PID 參數
    
    if isempty(xm_1)
        xm_1 = [0; 0; 0]; 
        xm_2 = [0; 0; 0];
        e_integral = [0; 0; 0];
        prev_error = [0; 0; 0];
        Kp = Kp_init; 
        Ki = Ki_init; 
        Kd = Kd_init;
    end
    
    % 初始化輸出變數
    u_vec = zeros(3,1);
    
    
    for i = 1:3
        
        % A. 參考模型動態
        u_model = wn_vec(i)^2 * cmd_vec(i);
        dxm_2 = -2*zeta_vec(i)*wn_vec(i)*xm_2(i) - wn_vec(i)^2*xm_1(i) + u_model;
        
        xm_2(i) = xm_2(i) + dxm_2 * dt;   % 速度積分
        xm_1(i) = xm_1(i) + xm_2(i) * dt; % 位置積分
        
        y_model = xm_1(i);
        
        % B. 誤差計算
        e_track = y_actual_vec(i) - y_model;  % 追蹤誤差
        e_ctrl  = cmd_vec(i) - y_actual_vec(i);   % 控制誤差
        
        % C. PID 訊號
        phi_p = e_ctrl;
        
        e_integral(i) = e_integral(i) + e_ctrl * dt;
        phi_i = e_integral(i);
        
        phi_d = (e_ctrl - prev_error(i)) / dt;
        prev_error(i) = e_ctrl;
        
        % D. Lyapunov 更新律
        dKp = -gam_p_vec(i) * e_track * phi_p;
        dKi = -gam_i_vec(i) * e_track * phi_i;
        dKd = -gam_d_vec(i) * e_track * phi_d;
        
        % 積分更新
        Kp(i) = Kp(i) + dKp * dt;
        Ki(i) = Ki(i) + dKi * dt;
        Kd(i) = Kd(i) + dKd * dt;
        
        % 參數限制
        Kp(i) = max(min(Kp(i), Kp_max(i)), Kp_min(i));
        Ki(i) = max(min(Ki(i), Ki_max(i)), Ki_min(i));
        Kd(i) = max(min(Kd(i), Kd_max(i)), Kd_min(i));
        
        % E. 計算控制力矩
        u_vec(i) = Kp(i)*phi_p + Ki(i)*phi_i + Kd(i)*phi_d;
    end
    
    % 輸出目前的 PID 參數
    K_log = [Kp; Ki; Kd]; 
end

== matlab function MRAC_PID_unblance_noposition/混合控制器/推力轉PWM ==
  data: force_N input; pwm_out output
function pwm_out = thrust2pwm(force_N)
   
    coeff_1 = [964.308, -21.41];  
    coeff_2 = [986.08, -217.69];
    coeff_3 = [958.89, -212.51];
    coeff_4 = [959.01, -210.12]; 

    % 整合係數矩陣
    Coeffs = [coeff_1; coeff_2; coeff_3; coeff_4];

    % 轉換邏輯
    pwm_out = zeros(4,1);
    g_gravity = 9.81;
    
    for i = 1:4
        % A. 牛頓轉公克
        thrust_g = (force_N(i) / g_gravity) * 1000;
        
        % B. 限制最小推力
        if thrust_g < 0
            thrust_g = 0;
        end
        
        % C. 反函數求解
        m = Coeffs(i, 1);
        c = Coeffs(i, 2);
        
        throttle_ratio = (thrust_g - c) / m;
        
        % D. 油門限制
        if throttle_ratio > 1
            throttle_ratio = 1;
        elseif throttle_ratio < 0
            throttle_ratio = 0; 
        end
        
        % E. 轉成 PWM
        % 1000 是怠速，1000 是範圍
        pwm_out(i) = 1000 + (throttle_ratio * 1000);
    end
end

== matlab function MRAC_PID_unblance_noposition/MATLAB Function ==
  data: States input; U input; d_States output; Pos output; Vel output; Angle output; Rate output; Ix input; Iy input; Iz input; az output
function [d_States, Pos, Vel, Angle, Rate,az] = DroneDynamics_ENU( States,U,Ix,Iy,Iz)


    % 1. 物理參數
    m = 2.0;            % 質量 (kg)
    g = 9.81;           % 重力 (m/s^2)
    
    % 慣量矩陣
    I = [Ix, 0, 0; 0, Iy, 0; 0, 0, Iz];
    I_inv = inv(I);

    % 2. 狀態解包
    % States = [x, y, z, vx, vy, vz, phi, theta, psi, p, q, r]
    x = States(1); y = States(2); z = States(3);
    % 速度
    vx = States(4); vy = States(5); vz = States(6);
    % 歐拉角
    phi = States(7); theta = States(8); psi = States(9);
    % 角速度
    p = States(10); q = States(11); r = States(12);

    % 3. 輸入解包
    % U = [Total_Thrust, Roll_Torque, Pitch_Torque, Yaw_Torque]
    F_thrust = U(1); % 總推力
    Tx = U(2);       % 滾轉力矩
    Ty = U(3);       % 俯仰力矩
    Tz = U(4);       % 偏航力矩
    Torque = [Tx; Ty; Tz];

    % 4. 旋轉矩陣

    cphi = cos(phi); sphi = sin(phi);
    cth = cos(theta); sth = sin(theta);
    cpsi = cos(psi); spsi = sin(psi);

    % 標準 ENU 旋轉矩陣
    R = [ cpsi*cth,  cpsi*sth*sphi - spsi*cphi,  cpsi*sth*cphi + spsi*sphi;
          spsi*cth,  spsi*sth*sphi + cpsi*cphi,  spsi*sth*cphi - cpsi*sphi;
             -sth,            cth*sphi,                  cth*cphi       ];

    % 5. 平移運動
    Thrust_body = [0; 0; F_thrust];
    
    % 轉換到地球座標系
    Forces_earth = R * Thrust_body;
    
    % 加入重力
    Gravity_earth = [0; 0; -m*g];
    % === 空氣阻力模型 (Air Drag) ===
    Cd = 0.3; 
    
    Drag_Force = -Cd * [vx; vy; vz];

    % 總加速度
    Acc_earth = (Forces_earth + Gravity_earth + Drag_Force) / m;
    
    ax = Acc_earth(1);
    ay = Acc_earth(2);
    az = Acc_earth(3);

    % 6. 旋轉運動    
    omega_body = [p; q; r];
    d_omega = I_inv * (Torque - cross(omega_body, I * omega_body));
    
    dp = d_omega(1);
    dq = d_omega(2);
    dr = d_omega(3);

    % 7. 運動學    
    % 變換矩陣 T
    % [dphi; dtheta; dpsi] = T * [p; q; r]
    tt = tan(theta);
    ct = cos(theta); 
    
    if abs(ct) < 1e-6 % 防止萬向節鎖死除以零
        ct = 1e-6;
    end
    sect = 1/ct;

    dphi   = p + q*sphi*tt + r*cphi*tt;
    dtheta =     q*cphi    - r*sphi;
    dpsi   =     q*sphi*sect + r*cphi*sect;

    % 8. 整合微分狀態
    d_States = [vx; vy; vz;      % d(Pos) = Vel
                ax; ay; az;      % d(Vel) = Acc
                dphi; dtheta; dpsi; % d(Angle)
                dp; dq; dr];     % d(Rate)
                
    % 9. 輸出監測
    Pos = [x; y; z];
    Vel = [vx; vy; vz];
    Angle = [phi; theta; psi];
    Rate = [p; q; r];
end

== matlab function MRAC_PID_unblance_noposition/Plant/PWM轉馬達推力 ==
  data: pwm_in input; force_N output
function force_N = pwm2thrust(pwm_in)


    Coeffs = [
        964.308, -21.41;   % M1
        986.08, -217.69;   % M2
        958.89, -212.51;   % M3
        959.01, -210.12    % M4
    ];

    force_N = zeros(4,1);
    g_gravity = 9.81;

    for i = 1:4
        % A. PWM 轉 油門比例
        throttle = (pwm_in(i) - 1000) / 1000;
        if throttle < 0, throttle = 0; end
        
        % B. 方程式
        m = Coeffs(i, 1);
        c = Coeffs(i, 2);
        
        thrust_g = m * throttle + c;
        
        % 物理限制
        if thrust_g < 0
            thrust_g = 0;
        end
        
        % C. 公克轉牛頓
        force_N(i) = (thrust_g / 1000) * g_gravity;
    end
end

== matlab function MRAC_PID_unblance_noposition/姿態估測器 ==
  data: roll_stick input; pitch_stick input; phi_cmd output; theta_cmd output; vx input; vy input
function [phi_cmd, theta_cmd] = XY_Logic_Controller(roll_stick, pitch_stick, vx, vy)

    deadzone = 0.1;        % 搖桿死區
    max_angle = 0.5;      % 最大飛行傾角
    brake_gain = 0.2;      % 煞車力道
    pitch_input = pitch_stick; 
    
    if abs(pitch_input) > deadzone
        theta_cmd = pitch_input * max_angle;
    else
        theta_cmd = (0 - vx) * brake_gain;
    end
    
    roll_input = -1 * roll_stick;
    
    if abs(roll_stick) > deadzone
        phi_cmd = roll_input * max_angle;
    else
        phi_cmd = (0 - vy) * brake_gain * -1;
    end
    
    % 安全限制
    limit = 0.5; 
    
    if theta_cmd > limit, theta_cmd = limit; end
    if theta_cmd < -limit, theta_cmd = -limit; end
    
    if phi_cmd > limit, phi_cmd = limit; end
    if phi_cmd < -limit, phi_cmd = -limit; end

end
